simulink model "ThermalLoop_draft3"  (R2024b)
settings: Solver=VariableStepAuto  StartTime=0.0  StopTime=2600
model workspace (MAT data in the model file):
  HX_HX = 500
  Kpipes = 14
  PumpHeat = 50
  TM_pipe = 50
libraries: fl_lib x28, nesl_utility x18, SimscapeFluids_lib x18, simulink x1
(part 2 of 2)

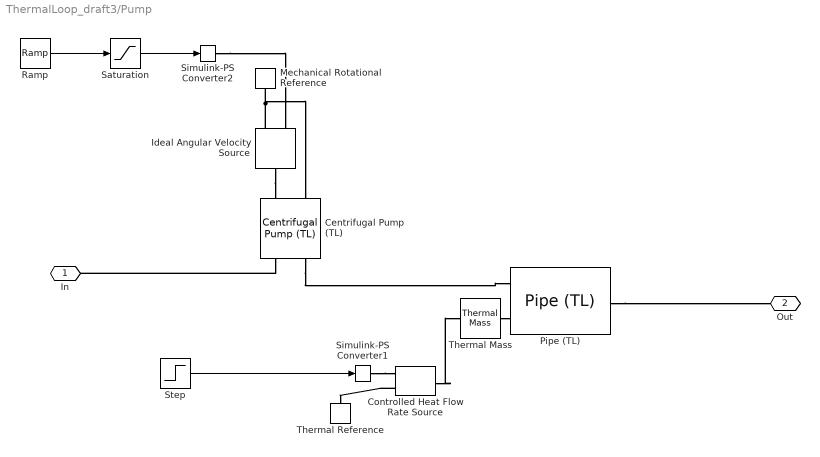
== system ThermalLoop_draft3/Pump ==
  Centrifugal Pump (TL) : SimscapeFluids_lib/Thermal Liquid/Pumps & Motors/Centrifugal Pump (TL)  pump_parameterization=fluids.thermal_liquid.pumps_motors.enum.CentrifugalPumpParameterization.Nominal  capacity_ref_nominal=15 gpm  head_ref_nominal=10 m  power_ref_nominal=0.85 kW  head_ref_max=20 m  capacity_ref_max=20 gpm  omega_ref_analytic=1770 rpm  flow_rate_1D_TLU=[16.67, 30, 40, 53.33, 66.67, 83.33] lpm  head_1D_TLU=[50, 47.5, 45, 40, 35, 25] m  power_1D_TLU=[.6, .75, .85, .93, .98, .99] kW  omega_ref_1D=3500 rpm  rho_ref_1D=998.21 kg/m^3  omega_threshold_factor=1e-2  flow_rate_2D_TLU=[16.67, 23.33, 30, 40, 53.33, 60] lpm  omega_2D_TLU=[2450, 2800, 3150, 3500] rpm  head_2D_TLU=[25, 32.7, 42.5, 50; 24, 31.7, 41, 49; 22.7, 30.5, 39, 47.5; 20, 28, 36, 45; 15.7, 24, 32, 40; 12.5, 21, 29.5, 37.5] m  power_2D_TLU=[.28, .38, .5, .6; .31, .41, .55, .68; .33, .44, .6, .75; .36, .48, .65, .83; .38, .53, .72, .93; .39, .55, .75, .97] kW  rho_ref_2D=998.21 kg/m^3  diameter_ratio=1  mech_orientation=fluids.thermal_liquid.pumps_motors.enum.CentrifugalPumpMechOrientation.Positive  area=4.52 in^2  operation_check=simscape.enum.assert.action.warn
      settings: InternalSimscapePortConfiguration="{\"Bottom\":[],\"Left\":[{\"id\":\"A\",\"label\":\"A\",\"type\":\"foundation.thermal_liquid.thermal_liquid\"},{\"id\":\"B\",\"label\":\"B\",\"type\":\"foundation.thermal_liquid.thermal_liquid\"}],\"Right\":[{\"id\":\"R\",\"label\":\"R\",\"type\":\"foundation.mechanical.rotational.rotational\"},{\"id\":\"C\",\"label\":\"C\",\"type\":\"foundation.mechanical.rotational.rotational\"}],\"Top\":[]}"
  Controlled Heat Flow Rate Source : fl_lib/Thermal/Thermal Sources/Controlled Heat Flow Rate Source
  Ideal Angular Velocity Source : fl_lib/Mechanical/Mechanical Sources/Ideal Angular Velocity Source
  Mechanical Rotational Reference : fl_lib/Mechanical/Rotational Elements/Mechanical Rotational Reference
  Pipe (TL) : SimscapeFluids_lib/Thermal Liquid/Pipes & Fittings/Pipe (TL)  dynamic_compressibility=true  inertia=false  num_segments=1  pipe_length=8 in  cross_section_geometry=fluids.thermal_liquid.pipes_fittings.enum.CrossSectionGeometry.Circular  pipe_diameter=2.4 in  pipe_inner_diameter=0.05 m  pipe_outer_diameter=0.1 m  pipe_width=0.1 m  pipe_height=0.1 m  pipe_major_axis=0.1 m  pipe_minor_axis=0.05 m  pipe_side=0.1 m  pipe_angle=30 deg  area=0.01 m^2  Dh=0.1128 m  elevation_spec=foundation.enum.constant_variable.constant  elevation_gain=0 m  gravity_spec=foundation.enum.constant_variable.constant  g=9.81 m/s^2  pressure_loss_spec=fluids.thermal_liquid.pipes_fittings.enum.PressureLossSpec.Haaland  local_pressure_loss_spec=fluids.thermal_liquid.pipes_fittings.enum.LocalLossSpec.AggregateLength  length_add=1 m  loss_coefficient=0.1  roughness_spec=fluids.thermal_liquid.pipes_fittings.enum.RoughnessSpec.SteelWroughtIron  roughness=15e-6 m  Re_friction_TLU=[400, 1000, 1500, 3000, 4000, 6000, 10000, 20000, 40000, 60000, 100000, 100000000]  friction_factor_TLU=[.264, .112, .071, .0417, .0387, .0268, .025, .0232, .0226, .022, .0214, .0214]  Re_lam=2000  Re_tur=4000  shape_factor=64  mdot_nominal=[.1, 1] kg/s  p_diff_nominal=[.001, .01] MPa  mdot_threshold=1e-6 kg/s  wall_spec=fluids.thermal_liquid.pipes_fittings.enum.wall_spec.rigid  vol_expansion_spec=fluids.thermal_liquid.pipes_fittings.enum.VolumeExpansionSpec.Area  area_pressure_gain=1e-6 m^2/MPa  static_pressure_TLU=[.1, 1] MPa  area_pressure_gain_TLU=[1e-05, 1.1e-05] m^2  material_behavior_spec=fluids.thermal_liquid.pipes_fittings.enum.PipeMaterialBehavior.Linear  diameter_pressure_gain=1e-6 m/MPa  wall_thickness=0.05 m  elastic_modulus=69 GPa  stress_TLU=[276, 310] MPa  strain_TLU=[.004, .02]  stress_assert_action=simscape.enum.assert.action.none  stress_max=400 MPa  poisson_ratio=0.33  wall_time_constant=0.01 s  thermal_expansion=false  alpha_L_wall=24 um/(deltaK*m)  thermal_expansion_Tref=293.15 K  heat_transfer_spec=fluids.thermal_liquid.pipes_fittings.enum.HeatTransferSpec.Gnielinski  mdot_nominal_heat=[.1, 1] kg/s  T_in_nominal=[293.15, 293.15] K  T_out_nominal=[300, 300] K  p_in_nominal_heat=[.101325, .101325] MPa  T_wall_nominal=[303.15, 303.15] K  a_coeff=0.023  b_Re_power=0.8  c_Pr_power=0.4  Nu_lam=3.66  Re_Colburn_TLU=[100, 150, 1000]  Colburn_factor_TLU=[.019, .013, .002]  Re_Nu_TLU=[100, 150, 1000]  Pr_Nu_TLU=[1, 10]  Nu_TLU=[3.72, 4.21; 3.75, 4.44; 4.21, 7.15]  p0_vec=0.101325 MPa  T0_vec=23 degC  mdot0=0.1 kg/s
  Ramp : simulink/Sources/Ramp  slope=1  start=1  InitialOutput=0
  Saturation : Saturate  UpperLimit=355  LowerLimit=0
  Simulink-PS Converter1 : nesl_utility/Simulink-PS Converter  PhysicalDomain=network_engine_domain  SubClassName=ps_input  LeftPortType=input  RightPortType=output  PseudoPeriodic=off  Frequencies=[]  NoiseDistribution=none  NoiseParameters=[]  Unit=W  AffineConversion=off  FilteringAndDerivatives=provide  SimscapeFilterOrder=1  InputFilterTimeConstant=0.001  UdotUserProvided=0
  Simulink-PS Converter2 : nesl_utility/Simulink-PS Converter  PhysicalDomain=network_engine_domain  SubClassName=ps_input  LeftPortType=input  RightPortType=output  PseudoPeriodic=off  Frequencies=[]  NoiseDistribution=none  NoiseParameters=[]  Unit=rad/s  AffineConversion=off  FilteringAndDerivatives=provide  SimscapeFilterOrder=1  InputFilterTimeConstant=0.001  UdotUserProvided=0
  Step : Step  Time=33  After=PumpHeat  SampleTime=0
  Thermal Mass : fl_lib/Thermal/Thermal Elements/Thermal Mass  mass_type=foundation.enum.constant_variable.constant  mass=1 kg  sp_heat=447 J/(K*kg)  mass_min=1e-6 kg  num_ports=foundation.enum.numPorts2.two  m_specify=off  m_priority=High  m=1 kg  m_nominal_specify=off  m_nominal_value=1  m_nominal_unit=kg  T_specify=on  T_priority=Low  T=297.15 K  T_nominal_specify=off  T_nominal_value=1  T_nominal_unit=K  Q_specify=off  Q_priority=None  Q=0 W  Q_nominal_specify=off  Q_nominal_value=1  Q_nominal_unit=W
      settings: InternalSimscapePortConfiguration="{\"Bottom\":[],\"Left\":[{\"id\":\"M\",\"label\":\"\",\"type\":\"foundation.thermal.thermal\"}],\"Right\":[{\"id\":\"N\",\"label\":\"\",\"type\":\"foundation.thermal.thermal\"}],\"Top\":[]}"
  Thermal Reference : fl_lib/Thermal/Thermal Elements/Thermal Reference
  In : PMIOPort  Side=Left
  Out : PMIOPort  Port=2  Side=Right
  wires:
  Step/1 -> Simulink-PS Converter1/1
  Saturation/1 -> Simulink-PS Converter2/1
  Ramp/1 -> Saturation/1
  connections:
  Centrifugal Pump (TL)/LConn1 -- In/RConn1
  Pipe (TL)/RConn1 -- Out/RConn1
  Thermal Mass/LConn1 -- Pipe (TL)/LConn2
  Simulink-PS Converter1/RConn1 -- Controlled Heat Flow Rate Source/RConn1
  Controlled Heat Flow Rate Source/RConn2 -- Thermal Reference/LConn1
  Controlled Heat Flow Rate Source/LConn1 -- Thermal Mass/RConn1
  Centrifugal Pump (TL)/LConn2 -- Pipe (TL)/LConn1
  Simulink-PS Converter2/RConn1 -- Ideal Angular Velocity Source/RConn1
  Ideal Angular Velocity Source/LConn1 -- Centrifugal Pump (TL)/RConn1
  Ideal Angular Velocity Source/RConn2 -- Centrifugal Pump (TL)/RConn2 -- Mechanical Rotational Reference/LConn1

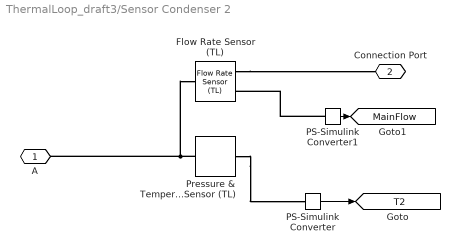
== system ThermalLoop_draft3/Sensor Condenser 2 ==
  Flow Rate Sensor (TL) : fl_lib/Thermal Liquid/Sensors/Flow Rate Sensor (TL)  mass_flow_measure=false  volumetric_flow_measure=true  energy_flow_measure=false
      settings: InternalSimscapePortConfiguration="{\"Bottom\":[],\"Left\":[{\"id\":\"A\",\"label\":\"A\",\"type\":\"foundation.thermal_liquid.thermal_liquid\"}],\"Right\":[{\"id\":\"B\",\"label\":\"B\",\"type\":\"foundation.thermal_liquid.thermal_liquid\"},{\"id\":\"V\",\"label\":\"V\",\"type\":\"output\"}],\"Top\":[]}"
  PS-Simulink Converter : nesl_utility/PS-Simulink Converter  PhysicalDomain=network_engine_domain  SubClassName=ps_output  LeftPortType=input  RightPortType=output  PseudoPeriodic=off  Frequencies=[]  VectorFormat=inherit  Unit=degC  AffineConversion=on
  PS-Simulink Converter1 : nesl_utility/PS-Simulink Converter  PhysicalDomain=network_engine_domain  SubClassName=ps_output  LeftPortType=input  RightPortType=output  PseudoPeriodic=off  Frequencies=[]  VectorFormat=inherit  Unit=gpm  AffineConversion=on
  Pressure & Temperature Sensor (TL) : fl_lib/Thermal Liquid/Sensors/Pressure & Temperature Sensor (TL)  reference=foundation.enum.MeasurementReference.absolute  pressure=false  pressure_spec=foundation.enum.PressureMeasementSpec.Absolute  temperature=true
      settings: InternalSimscapePortConfiguration="{\"Bottom\":[{\"id\":\"T\",\"label\":\"T\",\"type\":\"output\"}],\"Left\":[{\"id\":\"A\",\"label\":\"A\",\"type\":\"foundation.thermal_liquid.thermal_liquid\"}],\"Right\":[],\"Top\":[]}"
  A : PMIOPort  Side=Left
  Connection Port : PMIOPort  Port=2  Side=Left
  tag scope: MainFlow=global, T2=global
  wires:
  PS-Simulink Converter/1 -> [T2]
  PS-Simulink Converter1/1 -> [MainFlow]
  connections:
  Pressure & Temperature Sensor (TL)/LConn1 -- Flow Rate Sensor (TL)/LConn1 -- A/RConn1
  Pressure & Temperature Sensor (TL)/RConn1 -- PS-Simulink Converter/LConn1
  Flow Rate Sensor (TL)/RConn1 -- Connection Port/RConn1
  PS-Simulink Converter1/LConn1 -- Flow Rate Sensor (TL)/RConn2

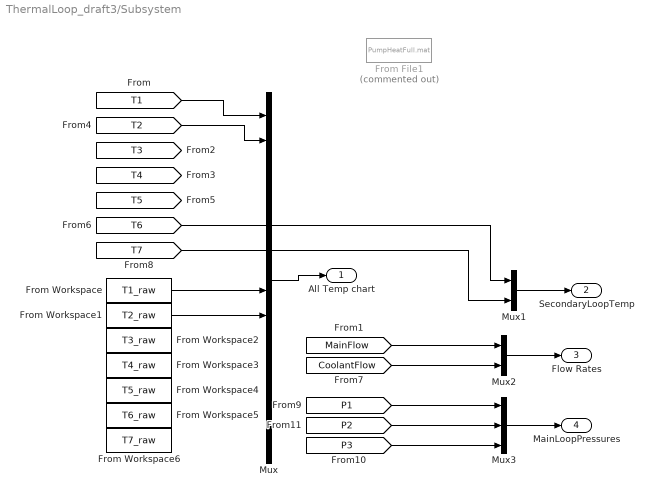
== system ThermalLoop_draft3/Subsystem ==
  From Workspace : FromWorkspace  VariableName=T1_raw  SampleTime=-1
  From Workspace1 : FromWorkspace  VariableName=T2_raw  SampleTime=-1
  From Workspace2 : FromWorkspace  VariableName=T3_raw  SampleTime=-1
  From Workspace3 : FromWorkspace  VariableName=T4_raw  SampleTime=-1
  From Workspace4 : FromWorkspace  VariableName=T5_raw  SampleTime=-1
  From Workspace5 : FromWorkspace  VariableName=T6_raw  SampleTime=-1
  From Workspace6 : FromWorkspace  VariableName=T7_raw  SampleTime=-1
  From File1 : FromFile  Commented=on  FileName=PumpHeatFull.mat  OutDataTypeStr=double  SampleTime=1
  Mux : Mux  Inputs=14
  Mux1 : Mux  Inputs=2
  Mux2 : Mux  Inputs=2
  Mux3 : Mux  Inputs=3
  All Temp chart : Outport
  SecondaryLoopTemp : Outport  Port=2
  Flow Rates : Outport  Port=3
  MainLoopPressures : Outport  Port=4
  wires:
  Mux/1 -> All Temp chart/1
  [T2] -> Mux/2
  [T1] -> Mux/1
  [MainFlow] -> Mux2/1
  [T7] -> Mux1/2
  Mux1/1 -> SecondaryLoopTemp/1
  [CoolantFlow] -> Mux2/2
  Mux2/1 -> Flow Rates/1
  Mux3/1 -> MainLoopPressures/1
  [P1] -> Mux3/1
  [P2] -> Mux3/2
  [P3] -> Mux3/3
  From Workspace/1 -> Mux/8
  From Workspace1/1 -> Mux/9
  [T6] -> Mux1/1

== system ThermalLoop_draft3/Thermocouple 2 ==
  PS-Simulink Converter : nesl_utility/PS-Simulink Converter  PhysicalDomain=network_engine_domain  SubClassName=ps_output  LeftPortType=input  RightPortType=output  PseudoPeriodic=off  Frequencies=[]  VectorFormat=inherit  Unit=degC  AffineConversion=on
  Pressure & Temperature Sensor (TL) : fl_lib/Thermal Liquid/Sensors/Pressure & Temperature Sensor (TL)  reference=foundation.enum.MeasurementReference.absolute  pressure=false  pressure_spec=foundation.enum.PressureMeasementSpec.Absolute  temperature=true
      settings: InternalSimscapePortConfiguration="{\"Bottom\":[{\"id\":\"T\",\"label\":\"T\",\"type\":\"output\"}],\"Left\":[{\"id\":\"A\",\"label\":\"A\",\"type\":\"foundation.thermal_liquid.thermal_liquid\"}],\"Right\":[],\"Top\":[]}"
  A : PMIOPort  Side=Left
  tag scope: T1=global
  wires:
  PS-Simulink Converter/1 -> [T1]
  connections:
  PS-Simulink Converter/LConn1 -- Pressure & Temperature Sensor (TL)/RConn1
  Pressure & Temperature Sensor (TL)/LConn1 -- A/RConn1

== system ThermalLoop_draft3/Ambient heat Losses/Thermocouple 1 ==
  PS-Simulink Converter : nesl_utility/PS-Simulink Converter  PhysicalDomain=network_engine_domain  SubClassName=ps_output  LeftPortType=input  RightPortType=output  PseudoPeriodic=off  Frequencies=[]  VectorFormat=inherit  Unit=degC  AffineConversion=on
  Temperature Sensor : fl_lib/Thermal/Thermal Sensors/Temperature Sensor  temperature_measure=foundation.enum.MeasurementReference.absolute
      settings: InternalSimscapePortConfiguration="{\"Bottom\":[],\"Left\":[{\"id\":\"A\",\"label\":\"A\",\"type\":\"foundation.thermal.thermal\"}],\"Right\":[{\"id\":\"T\",\"label\":\"T\",\"type\":\"output\"}],\"Top\":[]}"
  A : PMIOPort  Side=Left
  tag scope: T_Room=global
  wires:
  PS-Simulink Converter/1 -> [T_Room]
  connections:
  PS-Simulink Converter/LConn1 -- Temperature Sensor/RConn1
  A/RConn1 -- Temperature Sensor/LConn1

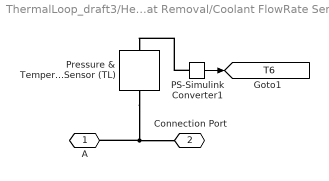
== system ThermalLoop_draft3/Heat Removal/Coolant FlowRate Sensor ==
  PS-Simulink Converter1 : nesl_utility/PS-Simulink Converter  PhysicalDomain=network_engine_domain  SubClassName=ps_output  LeftPortType=input  RightPortType=output  PseudoPeriodic=off  Frequencies=[]  VectorFormat=inherit  Unit=degC  AffineConversion=on
  Pressure & Temperature Sensor (TL) : fl_lib/Thermal Liquid/Sensors/Pressure & Temperature Sensor (TL)  reference=foundation.enum.MeasurementReference.absolute  pressure=false  pressure_spec=foundation.enum.PressureMeasementSpec.Absolute  temperature=true
      settings: InternalSimscapePortConfiguration="{\"Bottom\":[{\"id\":\"T\",\"label\":\"T\",\"type\":\"output\"}],\"Left\":[{\"id\":\"A\",\"label\":\"A\",\"type\":\"foundation.thermal_liquid.thermal_liquid\"}],\"Right\":[],\"Top\":[]}"
  A : PMIOPort  Side=Left
  Connection Port : PMIOPort  Port=2  Side=Right
  tag scope: T6=global
  wires:
  PS-Simulink Converter1/1 -> [T6]
  connections:
  Pressure & Temperature Sensor (TL)/LConn1 -- Connection Port/RConn1 -- A/RConn1
  PS-Simulink Converter1/LConn1 -- Pressure & Temperature Sensor (TL)/RConn1

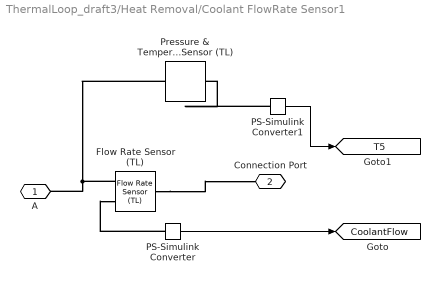
== system ThermalLoop_draft3/Heat Removal/Coolant FlowRate Sensor1 ==
  Flow Rate Sensor (TL) : fl_lib/Thermal Liquid/Sensors/Flow Rate Sensor (TL)  mass_flow_measure=false  volumetric_flow_measure=true  energy_flow_measure=false
      settings: InternalSimscapePortConfiguration="{\"Bottom\":[],\"Left\":[{\"id\":\"A\",\"label\":\"A\",\"type\":\"foundation.thermal_liquid.thermal_liquid\"}],\"Right\":[{\"id\":\"B\",\"label\":\"B\",\"type\":\"foundation.thermal_liquid.thermal_liquid\"},{\"id\":\"V\",\"label\":\"V\",\"type\":\"output\"}],\"Top\":[]}"
  PS-Simulink Converter : nesl_utility/PS-Simulink Converter  PhysicalDomain=network_engine_domain  SubClassName=ps_output  LeftPortType=input  RightPortType=output  PseudoPeriodic=off  Frequencies=[]  VectorFormat=inherit  Unit=gpm  AffineConversion=on
  PS-Simulink Converter1 : nesl_utility/PS-Simulink Converter  PhysicalDomain=network_engine_domain  SubClassName=ps_output  LeftPortType=input  RightPortType=output  PseudoPeriodic=off  Frequencies=[]  VectorFormat=inherit  Unit=degC  AffineConversion=on
  Pressure & Temperature Sensor (TL) : fl_lib/Thermal Liquid/Sensors/Pressure & Temperature Sensor (TL)  reference=foundation.enum.MeasurementReference.absolute  pressure=false  pressure_spec=foundation.enum.PressureMeasementSpec.Absolute  temperature=true
      settings: InternalSimscapePortConfiguration="{\"Bottom\":[{\"id\":\"T\",\"label\":\"T\",\"type\":\"output\"}],\"Left\":[{\"id\":\"A\",\"label\":\"A\",\"type\":\"foundation.thermal_liquid.thermal_liquid\"}],\"Right\":[],\"Top\":[]}"
  A : PMIOPort  Side=Left
  Connection Port : PMIOPort  Port=2  Side=Right
  tag scope: CoolantFlow=global, T5=global
  wires:
  PS-Simulink Converter/1 -> [CoolantFlow]
  PS-Simulink Converter1/1 -> [T5]
  connections:
  PS-Simulink Converter/LConn1 -- Flow Rate Sensor (TL)/RConn2
  Pressure & Temperature Sensor (TL)/LConn1 -- A/RConn1 -- Flow Rate Sensor (TL)/RConn1
  PS-Simulink Converter1/LConn1 -- Pressure & Temperature Sensor (TL)/RConn1
  Flow Rate Sensor (TL)/LConn1 -- Connection Port/RConn1
